simulink model "dclink2_ripple"  (R2026b)
settings: Solver=ode23tb  StopTime=1.2  MaxStep=Ts/4  RelTol=1e-6
values from neighbouring files (symbols this model uses):
  C = 40e-6    (= 4e-05)    [dclink2_ripple_params.m]    (also in resonant_example.m)
  fg = 50    [dclink2_ripple_params.m]
  iL0 = VbuckSet/Rload1    (= 10)    [dclink2_ripple_params.m]
  Kp = 1e-3    (= 0.001)    [dclink2_ripple_params.m]
  L = 220e-6    (= 0.00022)    [dclink2_ripple_params.m]    (also in resonant_example.m)
  m0 = (VbuckSet + RL*VbuckSet/R)/Vdc1    [bode_dclink2_ripple.m]    (also in dclink2_ripple_params.m = 0.7525; resonant_example.m = 0.7525)
  mMax = 0.95    [dclink2_ripple_params.m]
  mMin = 0    [dclink2_ripple_params.m]
  resA = zeros(2*nRes)    [resonant_example.m]
  resB = zeros(2*nRes, 1)    [resonant_example.m]
  resC = zeros(1, 2*nRes)    [resonant_example.m]
  resD = resD + b(k, 1)    [resonant_example.m]
  resEnable = 1    [dclink2_ripple_params.m]
  resGainScale = 1    [dclink2_ripple_params.m]
  RL = 0.1    [dclink2_ripple_params.m]    (also in resonant_example.m)
  Rload1 = Rnom    (= 30)    [dclink2_ripple_params.m]
  Rload2 = Rnom    (= 30)    [dclink2_ripple_params.m]
  Ts = 1/fCtrl    (= 0.000103447919145)    [dclink2_ripple_params.m]    (also in resonant_example.m)
  tStep = 0.6    [dclink2_ripple_params.m]
  VbuckSet = 300    [dclink2_ripple_params.m]
  vC0 = VbuckSet    (= 300)    [dclink2_ripple_params.m]
  Vdc1 = 400    [dclink2_ripple_params.m]    (also in resonant_example.m)
undefined symbols (not defined in the file or in its folder): DiscIntNeverNeededParam, notchDen, notchNum, ripAmp1, ripAmp2, ripH, ripPh1, ripPh2
settings Model: Creator=BenjaminRupp  LastModifiedBy=BenjaminRupp
settings DataIOCC: SaveOutput=off  SaveTime=off

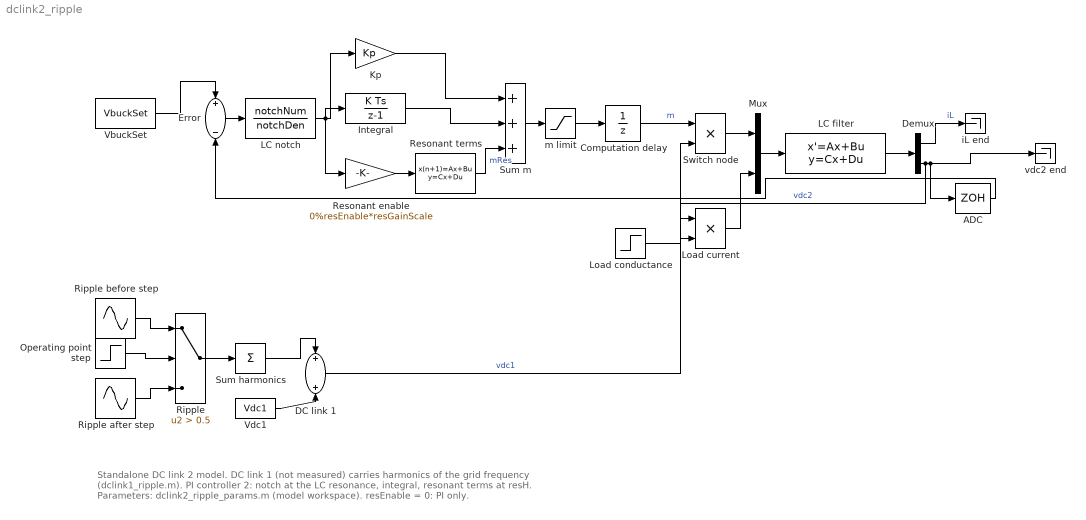
== system dclink2_ripple ==
  note: Standalone DC link 2 model. DC link 1 (not measured) carries harmonics of the grid
      | frequency (dclink1_ripple.m). PI controller 2: notch at the LC resonance, integral, resonant terms at resH.
      | Parameters: dclink2_ripple_params.m (model workspace). resEnable = 0: PI only.
  ADC : ZeroOrderHold  SampleTime=Ts
  Computation delay : UnitDelay  InitialCondition=m0  SampleTime=Ts
  DC link 1 : Sum
  Demux : Demux  Outputs=2
  Error : Sum  Inputs=+-
  Integral : DiscreteIntegrator  gainval=Ki  InitialCondition=m0  SampleTime=Ts  LimitOutput=on  UpperSaturationLimit=mMax  LowerSaturationLimit=mMin  ICPrevOutput=DiscIntNeverNeededParam  ICPrevScaledInput=DiscIntNeverNeededParam
  Kp : Gain  Gain=Kp
  LC filter : StateSpace  A=[-RL/L, -1/L; 1/C, 0]  B=[1/L, 0; 0, -1/C]  C=eye(2)  D=zeros(2)  InitialCondition=[iL0; vC0]
  LC notch : DiscreteTransferFcn  Numerator=notchNum  Denominator=notchDen  SampleTime=Ts
  Load conductance : Step  Time=tStep  InitialValue=1/Rload1  FinalValue=1/Rload2  SampleTime=0
  Load current : Product  Inputs=**
  Mux : Mux  Inputs=2
  Operating point step : Step  Time=tStep  SampleTime=0
  Resonant enable : Gain  Gain=0%resEnable*resGainScale
  Resonant terms : DiscreteStateSpace  Description=Sum over resH of Kr*(s*cos(th) - w*sin(th))/(s^2 + 2*wc*s + w^2), each Tustin prewarped at w (dclink2_resonant_coeffs.m)  A=resA  B=resB  C=resC  D=resD  SampleTime=Ts
  Ripple : Switch  Criteria=u2 > Threshold  Threshold=0.5  SaturateOnIntegerOverflow=off  InputSameDT=off
  Ripple after step : Sin  Amplitude=ripAmp2  Frequency=2*pi*fg*ripH  Phase=ripPh2  SampleTime=0
  Ripple before step : Sin  Amplitude=ripAmp1  Frequency=2*pi*fg*ripH  Phase=ripPh1  SampleTime=0
  Sum harmonics : Sum  Inputs=+
  Sum m : Sum  Inputs=+++
  Switch node : Product  Inputs=**
  VbuckSet : Constant  Value=VbuckSet
  Vdc1 : Constant  Value=Vdc1
  iL end : Terminator
  m limit : Saturate  UpperLimit=mMax  LowerLimit=mMin
  vdc2 end : Terminator
  wires:
  Ripple before step/1 -> Ripple/1
  Operating point step/1 -> Ripple/2
  Ripple after step/1 -> Ripple/3
  Ripple/1 -> Sum harmonics/1
  Sum harmonics/1 -> DC link 1/1
  Vdc1/1 -> DC link 1/2
  VbuckSet/1 -> Error/1
  ADC/1 -> Error/2
  Error/1 -> LC notch/1
  LC notch/1 -> Kp/1, Integral/1, Resonant enable/1
  Resonant enable/1 -> Resonant terms/1
  Kp/1 -> Sum m/1
  Integral/1 -> Sum m/2
  Resonant terms/1 -> Sum m/3  "mRes"
  Sum m/1 -> m limit/1
  m limit/1 -> Computation delay/1
  Computation delay/1 -> Switch node/1  "m"
  DC link 1/1 -> Switch node/2  "vdc1"
  Switch node/1 -> Mux/1
  Load current/1 -> Mux/2
  Mux/1 -> LC filter/1
  LC filter/1 -> Demux/1
  Demux/1 -> iL end/1  "iL"
  Demux/2 -> vdc2 end/1, ADC/1, Load current/1  "vdc2"
  Load conductance/1 -> Load current/2
